simulink model "sensor_BARO_model"  (R2025b)
settings: Solver=FixedStepDiscrete  StartTime=0.0  StopTime=20  FixedStep=0.001  RelTol=1e-3
undefined symbols (not defined in the file or in its folder): BARO_SAMPLE_RATE, IMU_SAMPLE_RATE
settings Model: DataDictionary=SensorDict.sldd  Creator=89447  LastModifiedBy=89447

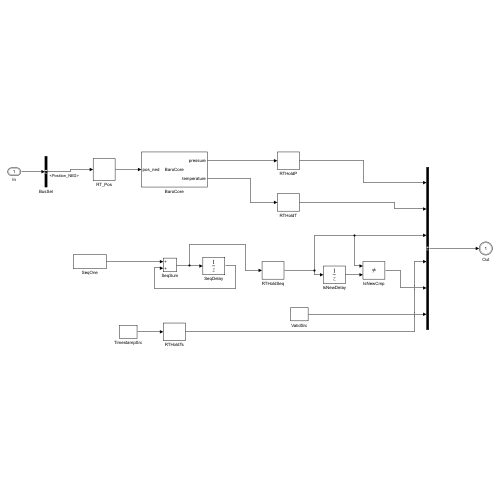
[thumbnail: Simulink's stored preview of the top-level diagram]
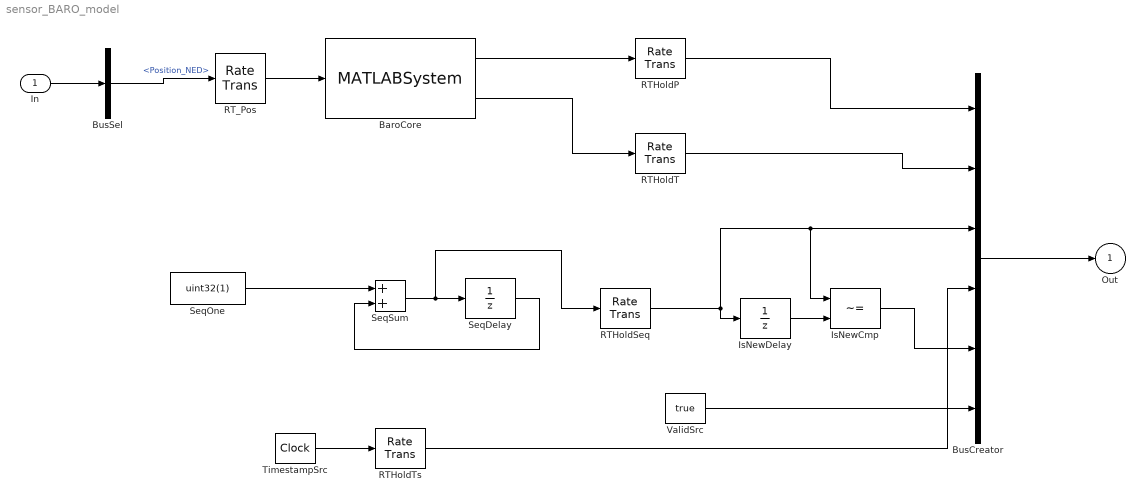
== system sensor_BARO_model ==
  In : Inport  OutDataTypeStr=Bus: DynamicModelBus
  BaroCore : MATLABSystem  System=BaroCore  SampleRate=50  ConstantBias=0  NoiseDensity=0  BiasInstability=0  DecayFactor=0  Seed=45601  RefAltMSL=0  TempOffset=0  TempNoise=0  LpfTau=0  RangeMin=0  RangeMax=1e12  Resolution=0  SimulateUsing=Interpreted execution
      mask Type: BaroCore
  BusCreator : BusCreator  Inputs=6  OutDataTypeStr=Bus: BarometerBus  NonVirtualBus=on
      settings: InheritFromInputs=off
  BusSel : BusSelector  OutputSignals=Position_NED
  IsNewCmp : RelationalOperator  Operator=~=  OutDataTypeStr=boolean  RndMeth=Simplest  InputSameDT=off
  IsNewDelay : UnitDelay  SampleTime=1/double(IMU_SAMPLE_RATE)  HasFrameUpgradeWarning=on
  RTHoldP : RateTransition  OutPortSampleTime=1/double(IMU_SAMPLE_RATE)
  RTHoldSeq : RateTransition  OutPortSampleTime=1/double(IMU_SAMPLE_RATE)
  RTHoldT : RateTransition  OutPortSampleTime=1/double(IMU_SAMPLE_RATE)
  RTHoldTs : RateTransition  OutPortSampleTime=1/double(IMU_SAMPLE_RATE)
  RT_Pos : RateTransition  OutPortSampleTime=1/double(BARO_SAMPLE_RATE)
  SeqDelay : UnitDelay  SampleTime=1/double(BARO_SAMPLE_RATE)  HasFrameUpgradeWarning=on
  SeqOne : Constant  Value=uint32(1)  OutDataTypeStr=uint32
  SeqSum : Sum  OutDataTypeStr=uint32
  TimestampSrc : DigitalClock  SampleTime=1/double(IMU_SAMPLE_RATE)
  ValidSrc : Constant  Value=true  OutDataTypeStr=boolean
  Out : Outport  OutDataTypeStr=Bus: BarometerBus
  wires:
  In/1 -> BusSel/1
  BusSel/1 -> RT_Pos/1  "<Position_NED>"
  RT_Pos/1 -> BaroCore/1
  BaroCore/1 -> RTHoldP/1
  BaroCore/2 -> RTHoldT/1
  RTHoldP/1 -> BusCreator/1
  RTHoldT/1 -> BusCreator/2
  SeqOne/1 -> SeqSum/1
  SeqDelay/1 -> SeqSum/2
  SeqSum/1 -> RTHoldSeq/1, SeqDelay/1
  RTHoldSeq/1 -> IsNewCmp/1, BusCreator/3, IsNewDelay/1
  IsNewDelay/1 -> IsNewCmp/2
  IsNewCmp/1 -> BusCreator/5
  TimestampSrc/1 -> RTHoldTs/1
  RTHoldTs/1 -> BusCreator/4
  ValidSrc/1 -> BusCreator/6
  BusCreator/1 -> Out/1
